simulink model "XY_Control"  (R2025b)
settings: Solver=FixedStepAuto  StartTime=0.0  StopTime=20  FixedStep=0.002  RelTol=1e-3  EnableMultiTasking=on
libraries: slpidlib x6, matrix_library x4, uavutilslib x1
settings Model: ExtModeTrigDuration=10000  Creator=plad  LastModifiedBy=David
settings SolverCC: AlgebraicLoopSolver=TrustRegion  PositivePriorityOrder=on
settings DataIOCC: ReturnWorkspaceOutputs=off
settings OptimizationCC: DefaultParameterBehavior=Inlined  EnhancedBackFolding=on  PassReuseOutputArgsAs=Individual arguments  ZeroExternalMemoryAtStartup=off  ZeroInternalMemoryAtStartup=off  MaxStackSize=64  OptimizeBlockOrder=speed  DifferentSizesBufferReuse=on  OptimizationCustomize=off  EfficientTunableParamExpr=on
settings DebuggingCC: ParameterTunabilityLossMsg=error  UnconnectedInputMsg=warning  UnconnectedOutputMsg=warning  UnconnectedLineMsg=warning  ArithmeticOperatorsInVariantConditions=warning
settings HardwareCC: ProdBitPerPointer=32.0  ProdBitPerSizeT=32.0  ProdBitPerPtrDiffT=32.0  ProdLargestAtomicFloat=None  ProdIntDivRoundTo=Undefined  ProdEndianess=Unspecified  ProdWordSize=32.0  ProdHWDeviceType=Generic->Unspecified (assume 32-bit Generic)
settings ModelReferenceCC: EnableRefExpFcnMdlSchedulingChecks=on
settings SFSimCC: SimUseLocalCustomCode=off  MATLABDynamicMemAlloc=off  CustomCodeUndefinedFunction=UseInterfaceOnly
settings RTWCC: SystemTargetFile=ert.tlc  TemplateMakefile=ert_default_tmf  RTWUseLocalCustomCode=off  TargetLang=C++  GPUComputeCapability=3.5  Description=Embedded Coder
settings CodeAppCC: ForceParamTrailComments=on  IgnoreCustomStorageClasses=off  OperatorAnnotations=on  SimulinkDataObjDesc=on  SFDataObjDesc=on  InsertBlockDesc=on
settings ERTTargetCC: ERTCustomFileTemplate=example_file_process.tlc
settings ConfigComp: CovMetricSettings=dswe

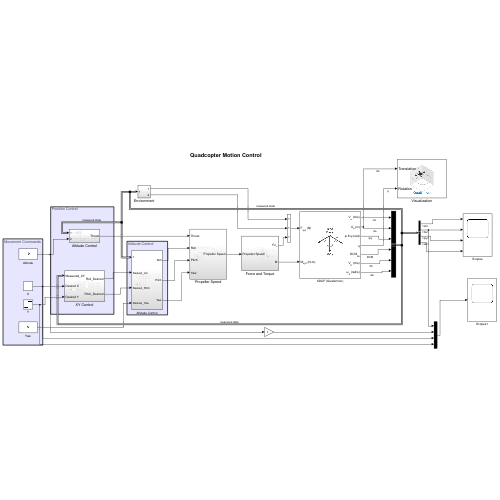
[thumbnail: Simulink's stored preview of the top-level diagram]
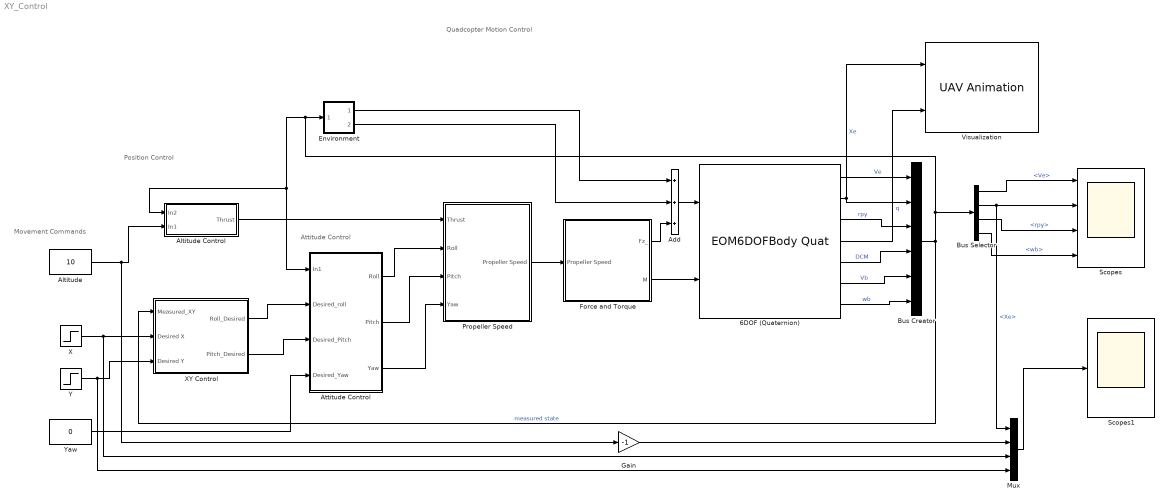
== system XY_Control ==
  note: Quadcopter Motion Control
  note: Attitude Control
  note: Position Control
  note: Movement Commands
  6DOF (Quaternion) : EOM6DOFBodyQuat
  Add : Sum  Inputs=+++
  Altitude : Constant  Value=10
  Altitude Control : Subsystem
  Attitude Control : Subsystem
  Bus Creator : BusCreator  Inputs=6
  Bus Selector : BusSelector  OutputSignals=Ve,Xe,rpy,wb
  Environment : Subsystem
  Force and Torque : Subsystem
  Gain : Gain  Gain=-1
  Mux : Mux
  Propeller Speed : Subsystem
  Scopes : Scope  NumInputPorts=4
      settings: ActiveDisplayYMinimum=-1  ActiveDisplayYMaximum=1
  Scopes1 : Scope
      settings: ActiveDisplayYMinimum=-65.352663287715231  ActiveDisplayYMaximum=14.57508700790809
  Visualization : uavutilslib/UAV Animation  NumUAV=1  DynamicUAVConfig=off  UAVType=Multirotor  UAVSize=1  UAVColor=[1 0 0]  UAVTrajectoryAlpha=1  InertialZDirection=Down  RotationFormat=Quaternion  DrawMarkers=off  SampleTime=-1
  X : Step  Time=3  After=4  SampleTime=0
  XY Control : Subsystem
  Y : Step  Time=3  After=8  SampleTime=0
  Yaw : Constant  Value=0
  wires:
  6DOF (Quaternion)/4 -> Visualization/2  "q"
  Altitude/1 -> Gain/1, Altitude Control/2(In1)
  X/1 -> Mux/3, XY Control/2(Desired X)
  Y/1 -> Mux/4, XY Control/3(Desired Y)
  XY Control/1(Roll_Desired) -> Attitude Control/2(Desired_roll)
  XY Control/2(Pitch_Desired) -> Attitude Control/3(Desired_Pitch)
  Yaw/1 -> Attitude Control/4(Desired_Yaw)
  Bus Creator/1 -> XY Control/1(Measured_XY), Attitude Control/1(In1), Altitude Control/1(In2), Environment/1(In1), Bus Selector/1  "measured state"
  Altitude Control/1(Thrust) -> Propeller Speed/1(Thrust)
  Attitude Control/1(Roll) -> Propeller Speed/2(Roll)
  Bus Selector/4 -> Scopes/4  "<wb>"
  Environment/1(Out1) -> Add/1
  Attitude Control/3(Yaw) -> Propeller Speed/4(Yaw)
  Attitude Control/2(Pitch) -> Propeller Speed/3(Pitch)
  Bus Selector/3 -> Scopes/3  "<rpy>"
  Bus Selector/1 -> Scopes/1  "<Ve>"
  Bus Selector/2 -> Scopes/2, Mux/1  "<Xe>"
  Environment/2(Out2) -> Add/2
  Propeller Speed/1(Propeller Speed) -> Force and Torque/1(Propeller Speed)
  Force and Torque/1(Fz_) -> Add/3
  6DOF (Quaternion)/2 -> Visualization/1, Bus Creator/2  "Xe"
  Add/1 -> 6DOF (Quaternion)/1
  Force and Torque/2(M) -> 6DOF (Quaternion)/2
  6DOF (Quaternion)/1 -> Bus Creator/1  "Ve"
  6DOF (Quaternion)/3 -> Bus Creator/3  "rpy"
  6DOF (Quaternion)/5 -> Bus Creator/4  "DCM"
  6DOF (Quaternion)/6 -> Bus Creator/5  "Vb"
  6DOF (Quaternion)/7 -> Bus Creator/6  "wb"
  Mux/1 -> Scopes1/1
  Gain/1 -> Mux/2

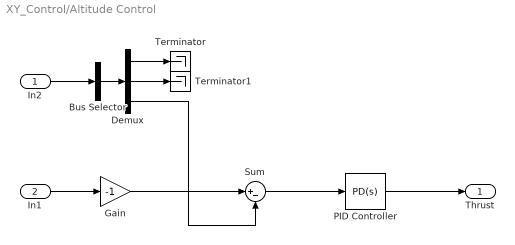
== system XY_Control/Altitude Control ==
  In2 : Inport
  In1 : Inport  Port=2
  Bus Selector : BusSelector  OutputSignals=Xe  OutputAsBus=on
  Demux : Demux  Outputs=3
  Gain : Gain  Gain=-1
  PID Controller : slpidlib/PID Controller  Controller=PD  Form=Parallel  TimeDomain=Continuous-time  UseExternalTs=off  SampleTime=-1  IntegratorMethod=Forward Euler  FilterMethod=Forward Euler  ControllerParametersSource=internal  P=1  I=1  UseKiTs=off  D=2  UseExternalDerivativeSource=off  N=100  UseFilter=on  TunerSelectOption=Transfer Function Based (PID Tuner App)  InitialConditionSource=internal  InitialConditionForIntegrator=0  InitialConditionForFilter=0  DifferentiatorICPrevScaledInput=0  ExternalReset=none  TrackingMode=off  Kt=1  LimitOutput=off  SatLimitsSource=internal  UpperSaturationLimit=inf  LowerSaturationLimit=-inf  LinearizeAsGain=on  AntiWindupMode=none  Kb=1  LimitIntegrator=off  UpperIntegratorSaturationLimit=inf  LowerIntegratorSaturationLimit=-inf  POutMin=[]  POutMax=[]  IOutMin=[]  IOutMax=[]  DOutMin=[]  DOutMax=[]  NOutMin=[]  NOutMax=[]  SumOutMin=[]  SumOutMax=[]  SaturationOutMin=[]  SaturationOutMax=[]  PParamMin=[]  PParamMax=[]  IParamMin=[]  IParamMax=[]  DParamMin=[]  DParamMax=[]  NParamMin=[]  NParamMax=[]  KbParamMin=[]  KbParamMax=[]  KtParamMin=[]  KtParamMax=[]  KbOutMin=[]  KbOutMax=[]  KtOutMin=[]  KtOutMax=[]  IntegratorOutMin=[]  IntegratorOutMax=[]  FilterOutMin=[]  FilterOutMax=[]  SumI1OutMin=[]  SumI1OutMax=[]  SumI2OutMin=[]  SumI2OutMax=[]  SumI3OutMin=[]  SumI3OutMax=[]  SumI4OutMin=[]  SumI4OutMax=[]  SumDOutMin=[]  SumDOutMax=[]  DifferentiatorOutMin=[]  DifferentiatorOutMax=[]  FilterDiffOutCoefMin=[]  FilterDiffOutCoefMax=[]  ReciprocalOutMin=[]  ReciprocalOutMax=[]  SumDenOutMin=[]  SumDenOutMax=[]  SumNumOutMin=[]  SumNumOutMax=[]  DivideOutMin=[]  DivideOutMax=[]  UdiffTsProdOutMin=[]  UdiffTsProdOutMax=[]  NTsProdOutMin=[]  NTsProdOutMax=[]  UintegralTsProdOutMin=[]  UintegralTsProdOutMax=[]  UngainTsProdOutMin=[]  UngainTsProdOutMax=[]  ClampingZeroOutDataTypeStr=Inherit: Inherit via back propagation  ClampingZeroOutMin=[]  ClampingZeroOutMax=[]  FilterDenConstantOutDataTypeStr=Inherit: Inherit via back propagation  FilterDenConstantOutMin=[]  FilterDenConstantOutMax=[]  PCopyOutDataTypeStr=Inherit: Inherit via back propagation  PCopyOutMin=[]  PCopyOutMax=[]  NCopyOutDataTypeStr=Inherit: Inherit via back propagation  NCopyOutMin=[]  NCopyOutMax=[]  IntegratorContinuousStateAttributes=''  IntegratorStateMustResolveToSignalObject=off  IntegratorRTWStateStorageClass=Auto  FilterContinuousStateAttributes=''  FilterStateMustResolveToSignalObject=off  FilterRTWStateStorageClass=Auto  ParallelPVariant=InternalParameters  IdealPVariant=Disabled  IVariant=Disabled  DVariant=InternalParameters  IntegratorVariant=Disabled  SatVariant=Disabled  AWVariant=Disabled  PCopyVariant=Disabled  TRVariant=Disabled  FdbkBlocksVariant=Forward  IdealPFdbkVariant=Disabled  SatFdbkVariant=Disabled  DerivativeFilterVariant=ContFilter  NVariant=InternalParameters  NCopyVariant=Disabled  FilterICVariant=InternalICsFilter  IntegratorICVariant=Disabled  ExternalResetVariant=Disabled  TRSumVariant=Passthrough  SumFdbkVariant=Disabled  SumVariant=Sum_PD  TsampFilterVariant=InternalTs  TsampNgainVariant=Passthrough  TsampIntegralVariant=Disabled_SignalSpec  ExternalSaturationOutDataTypeStr=Inherit: Same as second input  DerivativeSourceVariant=ErrorSignal  PreIntVariant=InternalPreInt
  Sum : Sum  Inputs=|+-
  Terminator : Terminator
  Terminator1 : Terminator
  Thrust : Outport
  wires:
  In2/1 -> Bus Selector/1
  Bus Selector/1 -> Demux/1
  Demux/2 -> Terminator1/1
  Demux/1 -> Terminator/1
  In1/1 -> Gain/1
  Demux/3 -> Sum/2
  Sum/1 -> PID Controller/1
  PID Controller/1 -> Thrust/1
  Gain/1 -> Sum/1

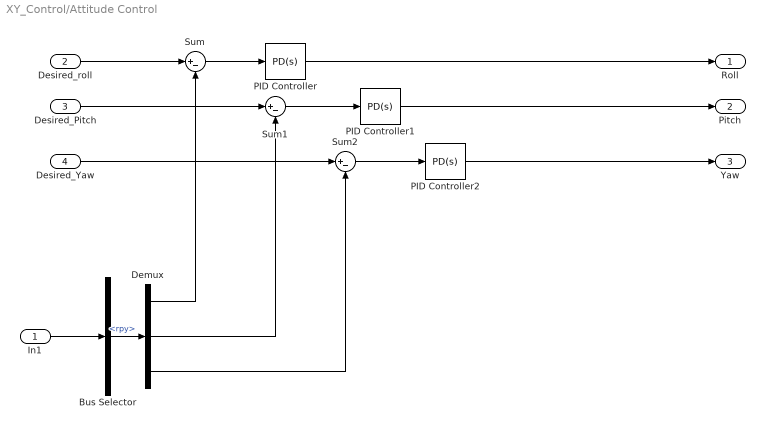
== system XY_Control/Attitude Control ==
  In1 : Inport
  Desired_roll : Inport  Port=2
  Desired_Pitch : Inport  Port=3
  Desired_Yaw : Inport  Port=4
  Bus Selector : BusSelector  OutputSignals=rpy
  Demux : Demux  Outputs=3
  PID Controller : slpidlib/PID Controller  Controller=PD  Form=Parallel  TimeDomain=Continuous-time  UseExternalTs=off  SampleTime=-1  IntegratorMethod=Forward Euler  FilterMethod=Forward Euler  ControllerParametersSource=internal  P=1  I=1  UseKiTs=off  D=2  UseExternalDerivativeSource=off  N=100  UseFilter=on  TunerSelectOption=Transfer Function Based (PID Tuner App)  InitialConditionSource=internal  InitialConditionForIntegrator=0  InitialConditionForFilter=0  DifferentiatorICPrevScaledInput=0  ExternalReset=none  TrackingMode=off  Kt=1  LimitOutput=off  SatLimitsSource=internal  UpperSaturationLimit=inf  LowerSaturationLimit=-inf  LinearizeAsGain=on  AntiWindupMode=none  Kb=1  LimitIntegrator=off  UpperIntegratorSaturationLimit=inf  LowerIntegratorSaturationLimit=-inf  POutMin=[]  POutMax=[]  IOutMin=[]  IOutMax=[]  DOutMin=[]  DOutMax=[]  NOutMin=[]  NOutMax=[]  SumOutMin=[]  SumOutMax=[]  SaturationOutMin=[]  SaturationOutMax=[]  PParamMin=[]  PParamMax=[]  IParamMin=[]  IParamMax=[]  DParamMin=[]  DParamMax=[]  NParamMin=[]  NParamMax=[]  KbParamMin=[]  KbParamMax=[]  KtParamMin=[]  KtParamMax=[]  KbOutMin=[]  KbOutMax=[]  KtOutMin=[]  KtOutMax=[]  IntegratorOutMin=[]  IntegratorOutMax=[]  FilterOutMin=[]  FilterOutMax=[]  SumI1OutMin=[]  SumI1OutMax=[]  SumI2OutMin=[]  SumI2OutMax=[]  SumI3OutMin=[]  SumI3OutMax=[]  SumI4OutMin=[]  SumI4OutMax=[]  SumDOutMin=[]  SumDOutMax=[]  DifferentiatorOutMin=[]  DifferentiatorOutMax=[]  FilterDiffOutCoefMin=[]  FilterDiffOutCoefMax=[]  ReciprocalOutMin=[]  ReciprocalOutMax=[]  SumDenOutMin=[]  SumDenOutMax=[]  SumNumOutMin=[]  SumNumOutMax=[]  DivideOutMin=[]  DivideOutMax=[]  UdiffTsProdOutMin=[]  UdiffTsProdOutMax=[]  NTsProdOutMin=[]  NTsProdOutMax=[]  UintegralTsProdOutMin=[]  UintegralTsProdOutMax=[]  UngainTsProdOutMin=[]  UngainTsProdOutMax=[]  ClampingZeroOutDataTypeStr=Inherit: Inherit via back propagation  ClampingZeroOutMin=[]  ClampingZeroOutMax=[]  FilterDenConstantOutDataTypeStr=Inherit: Inherit via back propagation  FilterDenConstantOutMin=[]  FilterDenConstantOutMax=[]  PCopyOutDataTypeStr=Inherit: Inherit via back propagation  PCopyOutMin=[]  PCopyOutMax=[]  NCopyOutDataTypeStr=Inherit: Inherit via back propagation  NCopyOutMin=[]  NCopyOutMax=[]  IntegratorContinuousStateAttributes=''  IntegratorStateMustResolveToSignalObject=off  IntegratorRTWStateStorageClass=Auto  FilterContinuousStateAttributes=''  FilterStateMustResolveToSignalObject=off  FilterRTWStateStorageClass=Auto  ParallelPVariant=InternalParameters  IdealPVariant=Disabled  IVariant=Disabled  DVariant=InternalParameters  IntegratorVariant=Disabled  SatVariant=Disabled  AWVariant=Disabled  PCopyVariant=Disabled  TRVariant=Disabled  FdbkBlocksVariant=Forward  IdealPFdbkVariant=Disabled  SatFdbkVariant=Disabled  DerivativeFilterVariant=ContFilter  NVariant=InternalParameters  NCopyVariant=Disabled  FilterICVariant=InternalICsFilter  IntegratorICVariant=Disabled  ExternalResetVariant=Disabled  TRSumVariant=Passthrough  SumFdbkVariant=Disabled  SumVariant=Sum_PD  TsampFilterVariant=InternalTs  TsampNgainVariant=Passthrough  TsampIntegralVariant=Disabled_SignalSpec  ExternalSaturationOutDataTypeStr=Inherit: Same as second input  DerivativeSourceVariant=ErrorSignal  PreIntVariant=InternalPreInt
  PID Controller1 : slpidlib/PID Controller  Controller=PD  Form=Parallel  TimeDomain=Continuous-time  UseExternalTs=off  SampleTime=-1  IntegratorMethod=Forward Euler  FilterMethod=Forward Euler  ControllerParametersSource=internal  P=1  I=1  UseKiTs=off  D=2  UseExternalDerivativeSource=off  N=100  UseFilter=on  TunerSelectOption=Transfer Function Based (PID Tuner App)  InitialConditionSource=internal  InitialConditionForIntegrator=0  InitialConditionForFilter=0  DifferentiatorICPrevScaledInput=0  ExternalReset=none  TrackingMode=off  Kt=1  LimitOutput=off  SatLimitsSource=internal  UpperSaturationLimit=inf  LowerSaturationLimit=-inf  LinearizeAsGain=on  AntiWindupMode=none  Kb=1  LimitIntegrator=off  UpperIntegratorSaturationLimit=inf  LowerIntegratorSaturationLimit=-inf  POutMin=[]  POutMax=[]  IOutMin=[]  IOutMax=[]  DOutMin=[]  DOutMax=[]  NOutMin=[]  NOutMax=[]  SumOutMin=[]  SumOutMax=[]  SaturationOutMin=[]  SaturationOutMax=[]  PParamMin=[]  PParamMax=[]  IParamMin=[]  IParamMax=[]  DParamMin=[]  DParamMax=[]  NParamMin=[]  NParamMax=[]  KbParamMin=[]  KbParamMax=[]  KtParamMin=[]  KtParamMax=[]  KbOutMin=[]  KbOutMax=[]  KtOutMin=[]  KtOutMax=[]  IntegratorOutMin=[]  IntegratorOutMax=[]  FilterOutMin=[]  FilterOutMax=[]  SumI1OutMin=[]  SumI1OutMax=[]  SumI2OutMin=[]  SumI2OutMax=[]  SumI3OutMin=[]  SumI3OutMax=[]  SumI4OutMin=[]  SumI4OutMax=[]  SumDOutMin=[]  SumDOutMax=[]  DifferentiatorOutMin=[]  DifferentiatorOutMax=[]  FilterDiffOutCoefMin=[]  FilterDiffOutCoefMax=[]  ReciprocalOutMin=[]  ReciprocalOutMax=[]  SumDenOutMin=[]  SumDenOutMax=[]  SumNumOutMin=[]  SumNumOutMax=[]  DivideOutMin=[]  DivideOutMax=[]  UdiffTsProdOutMin=[]  UdiffTsProdOutMax=[]  NTsProdOutMin=[]  NTsProdOutMax=[]  UintegralTsProdOutMin=[]  UintegralTsProdOutMax=[]  UngainTsProdOutMin=[]  UngainTsProdOutMax=[]  ClampingZeroOutDataTypeStr=Inherit: Inherit via back propagation  ClampingZeroOutMin=[]  ClampingZeroOutMax=[]  FilterDenConstantOutDataTypeStr=Inherit: Inherit via back propagation  FilterDenConstantOutMin=[]  FilterDenConstantOutMax=[]  PCopyOutDataTypeStr=Inherit: Inherit via back propagation  PCopyOutMin=[]  PCopyOutMax=[]  NCopyOutDataTypeStr=Inherit: Inherit via back propagation  NCopyOutMin=[]  NCopyOutMax=[]  IntegratorContinuousStateAttributes=''  IntegratorStateMustResolveToSignalObject=off  IntegratorRTWStateStorageClass=Auto  FilterContinuousStateAttributes=''  FilterStateMustResolveToSignalObject=off  FilterRTWStateStorageClass=Auto  ParallelPVariant=InternalParameters  IdealPVariant=Disabled  IVariant=Disabled  DVariant=InternalParameters  IntegratorVariant=Disabled  SatVariant=Disabled  AWVariant=Disabled  PCopyVariant=Disabled  TRVariant=Disabled  FdbkBlocksVariant=Forward  IdealPFdbkVariant=Disabled  SatFdbkVariant=Disabled  DerivativeFilterVariant=ContFilter  NVariant=InternalParameters  NCopyVariant=Disabled  FilterICVariant=InternalICsFilter  IntegratorICVariant=Disabled  ExternalResetVariant=Disabled  TRSumVariant=Passthrough  SumFdbkVariant=Disabled  SumVariant=Sum_PD  TsampFilterVariant=InternalTs  TsampNgainVariant=Passthrough  TsampIntegralVariant=Disabled_SignalSpec  ExternalSaturationOutDataTypeStr=Inherit: Same as second input  DerivativeSourceVariant=ErrorSignal  PreIntVariant=InternalPreInt
  PID Controller2 : slpidlib/PID Controller  Controller=PD  Form=Parallel  TimeDomain=Continuous-time  UseExternalTs=off  SampleTime=-1  IntegratorMethod=Forward Euler  FilterMethod=Forward Euler  ControllerParametersSource=internal  P=1  I=1  UseKiTs=off  D=2  UseExternalDerivativeSource=off  N=100  UseFilter=on  TunerSelectOption=Transfer Function Based (PID Tuner App)  InitialConditionSource=internal  InitialConditionForIntegrator=0  InitialConditionForFilter=0  DifferentiatorICPrevScaledInput=0  ExternalReset=none  TrackingMode=off  Kt=1  LimitOutput=off  SatLimitsSource=internal  UpperSaturationLimit=inf  LowerSaturationLimit=-inf  LinearizeAsGain=on  AntiWindupMode=none  Kb=1  LimitIntegrator=off  UpperIntegratorSaturationLimit=inf  LowerIntegratorSaturationLimit=-inf  POutMin=[]  POutMax=[]  IOutMin=[]  IOutMax=[]  DOutMin=[]  DOutMax=[]  NOutMin=[]  NOutMax=[]  SumOutMin=[]  SumOutMax=[]  SaturationOutMin=[]  SaturationOutMax=[]  PParamMin=[]  PParamMax=[]  IParamMin=[]  IParamMax=[]  DParamMin=[]  DParamMax=[]  NParamMin=[]  NParamMax=[]  KbParamMin=[]  KbParamMax=[]  KtParamMin=[]  KtParamMax=[]  KbOutMin=[]  KbOutMax=[]  KtOutMin=[]  KtOutMax=[]  IntegratorOutMin=[]  IntegratorOutMax=[]  FilterOutMin=[]  FilterOutMax=[]  SumI1OutMin=[]  SumI1OutMax=[]  SumI2OutMin=[]  SumI2OutMax=[]  SumI3OutMin=[]  SumI3OutMax=[]  SumI4OutMin=[]  SumI4OutMax=[]  SumDOutMin=[]  SumDOutMax=[]  DifferentiatorOutMin=[]  DifferentiatorOutMax=[]  FilterDiffOutCoefMin=[]  FilterDiffOutCoefMax=[]  ReciprocalOutMin=[]  ReciprocalOutMax=[]  SumDenOutMin=[]  SumDenOutMax=[]  SumNumOutMin=[]  SumNumOutMax=[]  DivideOutMin=[]  DivideOutMax=[]  UdiffTsProdOutMin=[]  UdiffTsProdOutMax=[]  NTsProdOutMin=[]  NTsProdOutMax=[]  UintegralTsProdOutMin=[]  UintegralTsProdOutMax=[]  UngainTsProdOutMin=[]  UngainTsProdOutMax=[]  ClampingZeroOutDataTypeStr=Inherit: Inherit via back propagation  ClampingZeroOutMin=[]  ClampingZeroOutMax=[]  FilterDenConstantOutDataTypeStr=Inherit: Inherit via back propagation  FilterDenConstantOutMin=[]  FilterDenConstantOutMax=[]  PCopyOutDataTypeStr=Inherit: Inherit via back propagation  PCopyOutMin=[]  PCopyOutMax=[]  NCopyOutDataTypeStr=Inherit: Inherit via back propagation  NCopyOutMin=[]  NCopyOutMax=[]  IntegratorContinuousStateAttributes=''  IntegratorStateMustResolveToSignalObject=off  IntegratorRTWStateStorageClass=Auto  FilterContinuousStateAttributes=''  FilterStateMustResolveToSignalObject=off  FilterRTWStateStorageClass=Auto  ParallelPVariant=InternalParameters  IdealPVariant=Disabled  IVariant=Disabled  DVariant=InternalParameters  IntegratorVariant=Disabled  SatVariant=Disabled  AWVariant=Disabled  PCopyVariant=Disabled  TRVariant=Disabled  FdbkBlocksVariant=Forward  IdealPFdbkVariant=Disabled  SatFdbkVariant=Disabled  DerivativeFilterVariant=ContFilter  NVariant=InternalParameters  NCopyVariant=Disabled  FilterICVariant=InternalICsFilter  IntegratorICVariant=Disabled  ExternalResetVariant=Disabled  TRSumVariant=Passthrough  SumFdbkVariant=Disabled  SumVariant=Sum_PD  TsampFilterVariant=InternalTs  TsampNgainVariant=Passthrough  TsampIntegralVariant=Disabled_SignalSpec  ExternalSaturationOutDataTypeStr=Inherit: Same as second input  DerivativeSourceVariant=ErrorSignal  PreIntVariant=InternalPreInt
  Sum : Sum  Inputs=|+-
  Sum1 : Sum  Inputs=|+-
  Sum2 : Sum  Inputs=|+-
  Roll : Outport
  Pitch : Outport  Port=2
  Yaw : Outport  Port=3
  wires:
  In1/1 -> Bus Selector/1
  Demux/3 -> Sum2/2
  Bus Selector/1 -> Demux/1  "<rpy>"
  Desired_roll/1 -> Sum/1
  Desired_Pitch/1 -> Sum1/1
  Desired_Yaw/1 -> Sum2/1
  Demux/1 -> Sum/2
  Demux/2 -> Sum1/2
  Sum/1 -> PID Controller/1
  PID Controller/1 -> Roll/1
  PID Controller1/1 -> Pitch/1
  Sum1/1 -> PID Controller1/1
  Sum2/1 -> PID Controller2/1
  PID Controller2/1 -> Yaw/1

== system XY_Control/Environment ==
  In1 : Inport
  Aerodynamic Drag : Subsystem
  Gravitational Force : Subsystem
  Out1 : Outport
  Out2 : Outport  Port=2
  wires:
  In1/1 -> Gravitational Force/1(In1), Aerodynamic Drag/1(In1)
  Aerodynamic Drag/1(Out1) -> Out1/1
  Gravitational Force/1(Out1) -> Out2/1

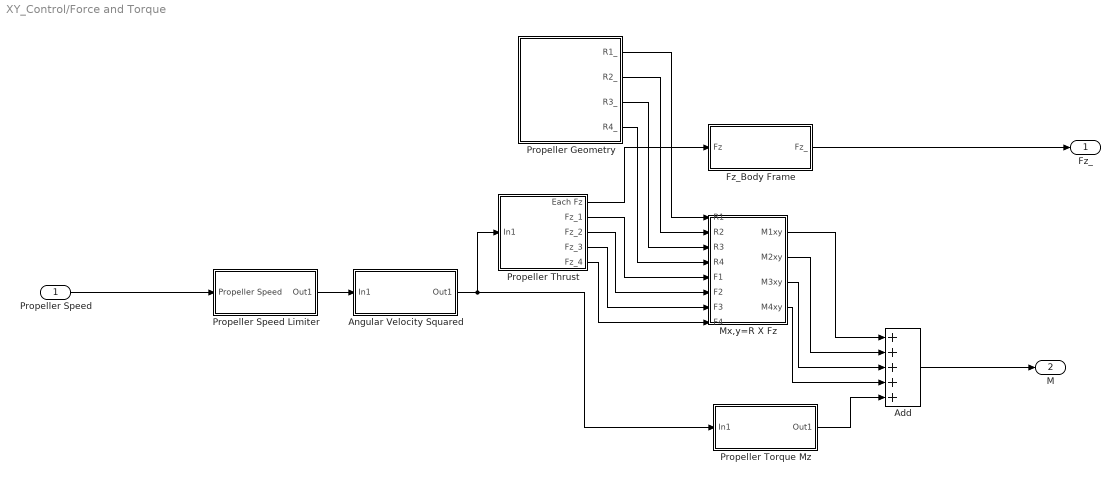
== system XY_Control/Force and Torque ==
  Propeller Speed : Inport
  Add : Sum  Inputs=+++++
  Angular Velocity Squared : Subsystem
  Fz_Body Frame : Subsystem
  Mx,y=R X Fz : Subsystem
  Propeller Geometry : Subsystem
  Propeller Speed Limiter : Subsystem
  Propeller Thrust : Subsystem
  Propeller Torque Mz : Subsystem
  Fz_ : Outport
  M : Outport  Port=2
  wires:
  Propeller Speed/1 -> Propeller Speed Limiter/1(Propeller Speed)
  Propeller Speed Limiter/1(Out1) -> Angular Velocity Squared/1(In1)
  Angular Velocity Squared/1(Out1) -> Propeller Torque Mz/1(In1), Propeller Thrust/1(In1)
  Add/1 -> M/1
  Propeller Torque Mz/1(Out1) -> Add/5
  Propeller Geometry/1(R1_) -> Mx,y=R X Fz/1(R1)
  Propeller Geometry/2(R2_) -> Mx,y=R X Fz/2(R2)
  Propeller Geometry/3(R3_) -> Mx,y=R X Fz/3(R3)
  Propeller Geometry/4(R4_) -> Mx,y=R X Fz/4(R4)
  Propeller Thrust/1(Each Fz) -> Fz_Body Frame/1(Fz)
  Propeller Thrust/2(Fz_1) -> Mx,y=R X Fz/5(F1)
  Propeller Thrust/3(Fz_2) -> Mx,y=R X Fz/6(F2)
  Propeller Thrust/4(Fz_3) -> Mx,y=R X Fz/7(F3)
  Propeller Thrust/5(Fz_4) -> Mx,y=R X Fz/8(F4)
  Fz_Body Frame/1(Fz_) -> Fz_/1
  Mx,y=R X Fz/1(M1xy) -> Add/1
  Mx,y=R X Fz/2(M2xy) -> Add/2
  Mx,y=R X Fz/3(M3xy) -> Add/3
  Mx,y=R X Fz/4(M4xy) -> Add/4

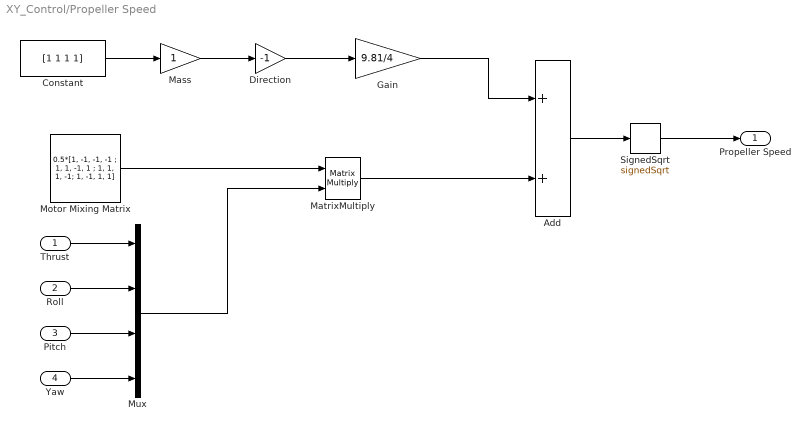
== system XY_Control/Propeller Speed ==
  Thrust : Inport
  Roll : Inport  Port=2
  Pitch : Inport  Port=3
  Yaw : Inport  Port=4
  Add : Sum
  Constant : Constant  Value=[1 1 1 1]
  Direction : Gain  Gain=-1
  Gain : Gain  Gain=9.81/4
  Mass : Gain
  MatrixMultiply : Product  Multiplication=Matrix(*)
  Motor Mixing Matrix : Constant  Value="0.5*[1, -1, -1, -1 ; 1, 1, -1, 1 ;   1, 1, 1, -1;  1, -1, 1, 1]"
  Mux : Mux
  SignedSqrt : Sqrt  Operator=signedSqrt  IntermediateResultsDataTypeStr=single
  Propeller Speed : Outport
  wires:
  Constant/1 -> Mass/1
  Mass/1 -> Direction/1
  Direction/1 -> Gain/1
  Gain/1 -> Add/1
  Thrust/1 -> Mux/1
  Roll/1 -> Mux/2
  Pitch/1 -> Mux/3
  Yaw/1 -> Mux/4
  Motor Mixing Matrix/1 -> MatrixMultiply/1
  Mux/1 -> MatrixMultiply/2
  MatrixMultiply/1 -> Add/2
  Add/1 -> SignedSqrt/1
  SignedSqrt/1 -> Propeller Speed/1

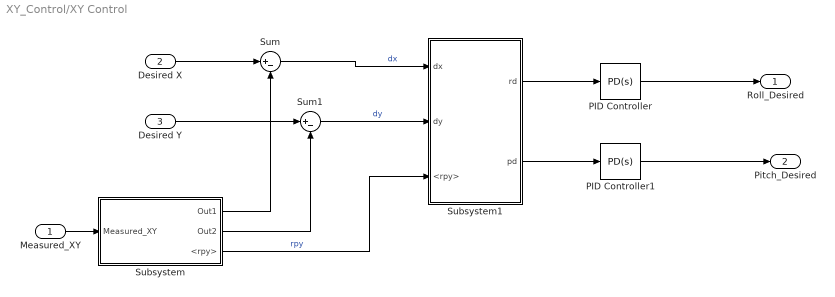
== system XY_Control/XY Control ==
  Measured_XY : Inport
  Desired X : Inport  Port=2
  Desired Y : Inport  Port=3
  PID Controller : slpidlib/PID Controller  Controller=PD  Form=Parallel  TimeDomain=Continuous-time  UseExternalTs=off  SampleTime=-1  IntegratorMethod=Forward Euler  FilterMethod=Forward Euler  ControllerParametersSource=internal  P=1  I=1  UseKiTs=off  D=2  UseExternalDerivativeSource=off  N=100  UseFilter=on  TunerSelectOption=Transfer Function Based (PID Tuner App)  InitialConditionSource=internal  InitialConditionForIntegrator=0  InitialConditionForFilter=0  DifferentiatorICPrevScaledInput=0  ExternalReset=none  TrackingMode=off  Kt=1  LimitOutput=on  SatLimitsSource=internal  UpperSaturationLimit=0.1  LowerSaturationLimit=-0.1  LinearizeAsGain=on  AntiWindupMode=none  Kb=1  LimitIntegrator=off  UpperIntegratorSaturationLimit=inf  LowerIntegratorSaturationLimit=-inf  POutMin=[]  POutMax=[]  IOutMin=[]  IOutMax=[]  DOutMin=[]  DOutMax=[]  NOutMin=[]  NOutMax=[]  SumOutMin=[]  SumOutMax=[]  SaturationOutMin=[]  SaturationOutMax=[]  PParamMin=[]  PParamMax=[]  IParamMin=[]  IParamMax=[]  DParamMin=[]  DParamMax=[]  NParamMin=[]  NParamMax=[]  KbParamMin=[]  KbParamMax=[]  KtParamMin=[]  KtParamMax=[]  KbOutMin=[]  KbOutMax=[]  KtOutMin=[]  KtOutMax=[]  IntegratorOutMin=[]  IntegratorOutMax=[]  FilterOutMin=[]  FilterOutMax=[]  SumI1OutMin=[]  SumI1OutMax=[]  SumI2OutMin=[]  SumI2OutMax=[]  SumI3OutMin=[]  SumI3OutMax=[]  SumI4OutMin=[]  SumI4OutMax=[]  SumDOutMin=[]  SumDOutMax=[]  DifferentiatorOutMin=[]  DifferentiatorOutMax=[]  FilterDiffOutCoefMin=[]  FilterDiffOutCoefMax=[]  ReciprocalOutMin=[]  ReciprocalOutMax=[]  SumDenOutMin=[]  SumDenOutMax=[]  SumNumOutMin=[]  SumNumOutMax=[]  DivideOutMin=[]  DivideOutMax=[]  UdiffTsProdOutMin=[]  UdiffTsProdOutMax=[]  NTsProdOutMin=[]  NTsProdOutMax=[]  UintegralTsProdOutMin=[]  UintegralTsProdOutMax=[]  UngainTsProdOutMin=[]  UngainTsProdOutMax=[]  ClampingZeroOutDataTypeStr=Inherit: Inherit via back propagation  ClampingZeroOutMin=[]  ClampingZeroOutMax=[]  FilterDenConstantOutDataTypeStr=Inherit: Inherit via back propagation  FilterDenConstantOutMin=[]  FilterDenConstantOutMax=[]  PCopyOutDataTypeStr=Inherit: Inherit via back propagation  PCopyOutMin=[]  PCopyOutMax=[]  NCopyOutDataTypeStr=Inherit: Inherit via back propagation  NCopyOutMin=[]  NCopyOutMax=[]  IntegratorContinuousStateAttributes=''  IntegratorStateMustResolveToSignalObject=off  IntegratorRTWStateStorageClass=Auto  FilterContinuousStateAttributes=''  FilterStateMustResolveToSignalObject=off  FilterRTWStateStorageClass=Auto  ParallelPVariant=InternalParameters  IdealPVariant=Disabled  IVariant=Disabled  DVariant=InternalParameters  IntegratorVariant=Disabled  SatVariant=Enabled  AWVariant=Disabled  PCopyVariant=Disabled  TRVariant=Disabled  FdbkBlocksVariant=Forward  IdealPFdbkVariant=Disabled  SatFdbkVariant=Disabled  DerivativeFilterVariant=ContFilter  NVariant=InternalParameters  NCopyVariant=Disabled  FilterICVariant=InternalICsFilter  IntegratorICVariant=Disabled  ExternalResetVariant=Disabled  TRSumVariant=Passthrough  SumFdbkVariant=Disabled  SumVariant=Sum_PD  TsampFilterVariant=InternalTs  TsampNgainVariant=Passthrough  TsampIntegralVariant=Disabled_SignalSpec  ExternalSaturationOutDataTypeStr=Inherit: Same as second input  DerivativeSourceVariant=ErrorSignal  PreIntVariant=InternalPreInt
  PID Controller1 : slpidlib/PID Controller  Controller=PD  Form=Parallel  TimeDomain=Continuous-time  UseExternalTs=off  SampleTime=-1  IntegratorMethod=Forward Euler  FilterMethod=Forward Euler  ControllerParametersSource=internal  P=1  I=1  UseKiTs=off  D=2  UseExternalDerivativeSource=off  N=100  UseFilter=on  TunerSelectOption=Frequency Response Based  InitialConditionSource=internal  InitialConditionForIntegrator=0  InitialConditionForFilter=0  DifferentiatorICPrevScaledInput=0  ExternalReset=none  TrackingMode=off  Kt=1  LimitOutput=on  SatLimitsSource=internal  UpperSaturationLimit=0.1  LowerSaturationLimit=-0.1  LinearizeAsGain=on  AntiWindupMode=none  Kb=1  LimitIntegrator=off  UpperIntegratorSaturationLimit=inf  LowerIntegratorSaturationLimit=-inf  POutMin=[]  POutMax=[]  IOutMin=[]  IOutMax=[]  DOutMin=[]  DOutMax=[]  NOutMin=[]  NOutMax=[]  SumOutMin=[]  SumOutMax=[]  SaturationOutMin=[]  SaturationOutMax=[]  PParamMin=[]  PParamMax=[]  IParamMin=[]  IParamMax=[]  DParamMin=[]  DParamMax=[]  NParamMin=[]  NParamMax=[]  KbParamMin=[]  KbParamMax=[]  KtParamMin=[]  KtParamMax=[]  KbOutMin=[]  KbOutMax=[]  KtOutMin=[]  KtOutMax=[]  IntegratorOutMin=[]  IntegratorOutMax=[]  FilterOutMin=[]  FilterOutMax=[]  SumI1OutMin=[]  SumI1OutMax=[]  SumI2OutMin=[]  SumI2OutMax=[]  SumI3OutMin=[]  SumI3OutMax=[]  SumI4OutMin=[]  SumI4OutMax=[]  SumDOutMin=[]  SumDOutMax=[]  DifferentiatorOutMin=[]  DifferentiatorOutMax=[]  FilterDiffOutCoefMin=[]  FilterDiffOutCoefMax=[]  ReciprocalOutMin=[]  ReciprocalOutMax=[]  SumDenOutMin=[]  SumDenOutMax=[]  SumNumOutMin=[]  SumNumOutMax=[]  DivideOutMin=[]  DivideOutMax=[]  UdiffTsProdOutMin=[]  UdiffTsProdOutMax=[]  NTsProdOutMin=[]  NTsProdOutMax=[]  UintegralTsProdOutMin=[]  UintegralTsProdOutMax=[]  UngainTsProdOutMin=[]  UngainTsProdOutMax=[]  ClampingZeroOutDataTypeStr=Inherit: Inherit via back propagation  ClampingZeroOutMin=[]  ClampingZeroOutMax=[]  FilterDenConstantOutDataTypeStr=Inherit: Inherit via back propagation  FilterDenConstantOutMin=[]  FilterDenConstantOutMax=[]  PCopyOutDataTypeStr=Inherit: Inherit via back propagation  PCopyOutMin=[]  PCopyOutMax=[]  NCopyOutDataTypeStr=Inherit: Inherit via back propagation  NCopyOutMin=[]  NCopyOutMax=[]  IntegratorContinuousStateAttributes=''  IntegratorStateMustResolveToSignalObject=off  IntegratorRTWStateStorageClass=Auto  FilterContinuousStateAttributes=''  FilterStateMustResolveToSignalObject=off  FilterRTWStateStorageClass=Auto  ParallelPVariant=InternalParameters  IdealPVariant=Disabled  IVariant=Disabled  DVariant=InternalParameters  IntegratorVariant=Disabled  SatVariant=Enabled  AWVariant=Disabled  PCopyVariant=Disabled  TRVariant=Disabled  FdbkBlocksVariant=Forward  IdealPFdbkVariant=Disabled  SatFdbkVariant=Disabled  DerivativeFilterVariant=ContFilter  NVariant=InternalParameters  NCopyVariant=Disabled  FilterICVariant=InternalICsFilter  IntegratorICVariant=Disabled  ExternalResetVariant=Disabled  TRSumVariant=Passthrough  SumFdbkVariant=Disabled  SumVariant=Sum_PD  TsampFilterVariant=InternalTs  TsampNgainVariant=Passthrough  TsampIntegralVariant=Disabled_SignalSpec  ExternalSaturationOutDataTypeStr=Inherit: Same as second input  DerivativeSourceVariant=ErrorSignal  PreIntVariant=InternalPreInt
  Subsystem : Subsystem
  Subsystem1 : Subsystem
  Sum : Sum  Inputs=|+-
  Sum1 : Sum  Inputs=|+-
  Roll_Desired : Outport
  Pitch_Desired : Outport  Port=2
  wires:
  Measured_XY/1 -> Subsystem/1(Measured_XY)
  Subsystem/1(Out1) -> Sum/2
  Subsystem/2(Out2) -> Sum1/2
  Desired X/1 -> Sum/1
  Desired Y/1 -> Sum1/1
  Sum/1 -> Subsystem1/1(dx)  "dx"
  Sum1/1 -> Subsystem1/2(dy)  "dy"
  Subsystem/3(<rpy>) -> Subsystem1/3(<rpy>)  "rpy"
  Subsystem1/2(pd) -> PID Controller1/1
  Subsystem1/1(rd) -> PID Controller/1
  PID Controller/1 -> Roll_Desired/1
  PID Controller1/1 -> Pitch_Desired/1

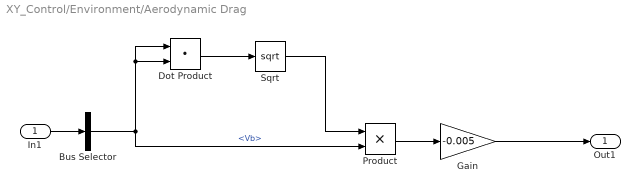
== system XY_Control/Environment/Aerodynamic Drag ==
  In1 : Inport
  Bus Selector : BusSelector  OutputSignals=Vb
  Dot Product : DotProduct  OutDataTypeStr=Inherit: Inherit via internal rule
  Gain : Gain  Gain=-0.005
  Product : Product
  Sqrt : Sqrt
  Out1 : Outport
  wires:
  In1/1 -> Bus Selector/1
  Bus Selector/1 -> Dot Product/1, Dot Product/2, Product/2  "<Vb>"
  Dot Product/1 -> Sqrt/1
  Sqrt/1 -> Product/1
  Product/1 -> Gain/1
  Gain/1 -> Out1/1

== system XY_Control/Environment/Gravitational Force ==
  In1 : Inport
  Gravitational Acceleration : Subsystem
  Mass : Gain
  Out1 : Outport
  wires:
  In1/1 -> Gravitational Acceleration/1(In1)
  Gravitational Acceleration/1(Out2) -> Mass/1
  Mass/1 -> Out1/1

== system XY_Control/Force and Torque/Angular Velocity Squared ==
  In1 : Inport
  Abs : Abs  SaturateOnIntegerOverflow=off
  Product : Product
  Out1 : Outport
  wires:
  Abs/1 -> Product/1
  Product/1 -> Out1/1
  In1/1 -> Product/2, Abs/1

== system XY_Control/Force and Torque/Fz_Body Frame ==
  Fz : Inport
  Sum of Elements : Sum  Inputs=+
  z-vector : Subsystem
  Fz_ : Outport
  wires:
  Fz/1 -> Sum of Elements/1
  z-vector/1(Fz_out) -> Fz_/1
  Sum of Elements/1 -> z-vector/1(Fz_in)

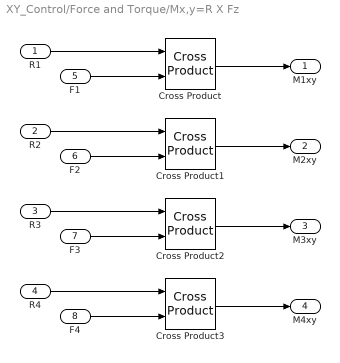
== system XY_Control/Force and Torque/Mx,y=R X Fz ==
  R1 : Inport
  R2 : Inport  Port=2
  R3 : Inport  Port=3
  R4 : Inport  Port=4
  F1 : Inport  Port=5
  F2 : Inport  Port=6
  F3 : Inport  Port=7
  F4 : Inport  Port=8
  Cross Product{,1..3} (4 alike) : matrix_library/Cross Product
  M1xy : Outport
  M2xy : Outport  Port=2
  M3xy : Outport  Port=3
  M4xy : Outport  Port=4
  wires:
  R1/1 -> Cross Product/1
  F1/1 -> Cross Product/2
  R2/1 -> Cross Product1/1
  F2/1 -> Cross Product1/2
  R3/1 -> Cross Product2/1
  F3/1 -> Cross Product2/2
  R4/1 -> Cross Product3/1
  F4/1 -> Cross Product3/2
  Cross Product/1 -> M1xy/1
  Cross Product1/1 -> M2xy/1
  Cross Product2/1 -> M3xy/1
  Cross Product3/1 -> M4xy/1

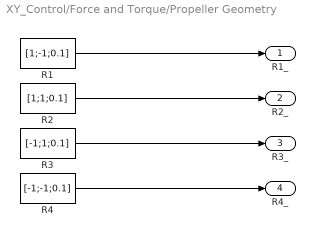
== system XY_Control/Force and Torque/Propeller Geometry ==
  R1 : Constant  Value=[1;-1;0.1]
  R2 : Constant  Value=[1;1;0.1]
  R3 : Constant  Value=[-1;1;0.1]
  R4 : Constant  Value=[-1;-1;0.1]
  R1_ : Outport
  R2_ : Outport  Port=2
  R3_ : Outport  Port=3
  R4_ : Outport  Port=4
  wires:
  R1/1 -> R1_/1
  R2/1 -> R2_/1
  R3/1 -> R3_/1
  R4/1 -> R4_/1

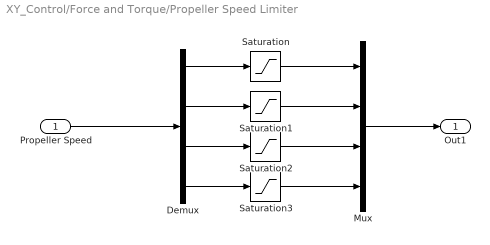
== system XY_Control/Force and Torque/Propeller Speed Limiter ==
  Propeller Speed : Inport
  Demux : Demux
  Mux : Mux
  Saturation{,1..3} (4 alike) : Saturate  UpperLimit=300  LowerLimit=-300
  Out1 : Outport
  wires:
  Propeller Speed/1 -> Demux/1
  Demux/1 -> Saturation/1
  Saturation/1 -> Mux/1
  Demux/2 -> Saturation1/1
  Demux/3 -> Saturation2/1
  Demux/4 -> Saturation3/1
  Saturation1/1 -> Mux/2
  Saturation2/1 -> Mux/3
  Saturation3/1 -> Mux/4
  Mux/1 -> Out1/1

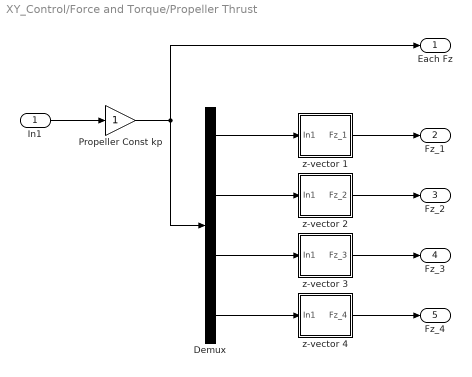
== system XY_Control/Force and Torque/Propeller Thrust ==
  In1 : Inport
  Demux : Demux
  Propeller Const kp : Gain
  z-vector 1 : Subsystem
  z-vector 2 : Subsystem
  z-vector 3 : Subsystem
  z-vector 4 : Subsystem
  Each Fz : Outport
  Fz_1 : Outport  Port=2
  Fz_2 : Outport  Port=3
  Fz_3 : Outport  Port=4
  Fz_4 : Outport  Port=5
  wires:
  In1/1 -> Propeller Const kp/1
  Propeller Const kp/1 -> Demux/1, Each Fz/1
  Demux/1 -> z-vector 1/1(In1)
  Demux/2 -> z-vector 2/1(In1)
  Demux/3 -> z-vector 3/1(In1)
  Demux/4 -> z-vector 4/1(In1)
  z-vector 1/1(Fz_1) -> Fz_1/1
  z-vector 2/1(Fz_2) -> Fz_2/1
  z-vector 3/1(Fz_3) -> Fz_3/1
  z-vector 4/1(Fz_4) -> Fz_4/1

== system XY_Control/Force and Torque/Propeller Torque Mz ==
  In1 : Inport
  Motor Torq Const km : Gain
  Subsystem : Subsystem
  Subsystem1 : Subsystem
  Out1 : Outport
  wires:
  In1/1 -> Motor Torq Const km/1
  Motor Torq Const km/1 -> Subsystem/1(In1)
  Subsystem/1(Out1) -> Subsystem1/1(In1)
  Subsystem1/1(Out1) -> Out1/1

== system XY_Control/XY Control/Subsystem ==
  Measured_XY : Inport
  Bus Selector : BusSelector  OutputSignals=Xe,rpy
  Demux : Demux  Outputs=3
  Terminator : Terminator
  Out1 : Outport
  Out2 : Outport  Port=2
  <rpy> : Outport  Port=3
  wires:
  Demux/3 -> Terminator/1
  Demux/2 -> Out2/1
  Measured_XY/1 -> Bus Selector/1
  Bus Selector/2 -> <rpy>/1  "<rpy>"
  Bus Selector/1 -> Demux/1  "<Xe>"
  Demux/1 -> Out1/1

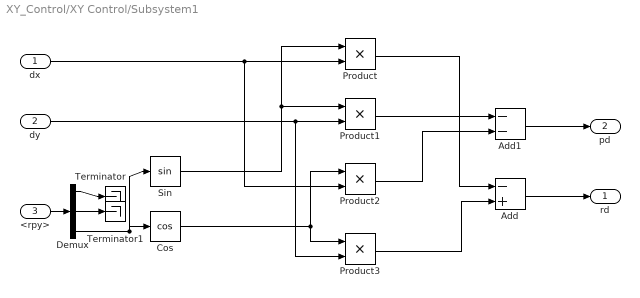
== system XY_Control/XY Control/Subsystem1 ==
  dx : Inport
  dy : Inport  Port=2
  <rpy> : Inport  Port=3
  Add : Sum  Inputs=-+
  Add1 : Sum  Inputs=--
  Cos : Trigonometry  Operator=cos
  Demux : Demux  Outputs=3
  Product{,1..3} (4 alike) : Product
  Sin : Trigonometry
  Terminator : Terminator
  Terminator1 : Terminator
  rd : Outport
  pd : Outport  Port=2
  wires:
  <rpy>/1 -> Demux/1
  Demux/1 -> Terminator/1
  Demux/2 -> Terminator1/1
  Demux/3 -> Cos/1, Sin/1
  Sin/1 -> Product/1, Product1/1
  dx/1 -> Product2/2, Product/2
  Product/1 -> Add/1
  Add/1 -> rd/1
  dy/1 -> Product3/2, Product1/2
  Product1/1 -> Add1/1
  Cos/1 -> Product3/1, Product2/1
  Product2/1 -> Add1/2
  Product3/1 -> Add/2
  Add1/1 -> pd/1

== system XY_Control/Environment/Gravitational Force/Gravitational Acceleration ==
  In1 : Inport
  Bus Selector1 : BusSelector  OutputSignals=DCM
  Constant2 : Constant  Value=[0;0;9.81]
  MatrixMultiply : Product  Multiplication=Matrix(*)
  Out2 : Outport
  wires:
  In1/1 -> Bus Selector1/1
  Bus Selector1/1 -> MatrixMultiply/1  "<DCM>"
  Constant2/1 -> MatrixMultiply/2
  MatrixMultiply/1 -> Out2/1

== system XY_Control/Force and Torque/Fz_Body Frame/z-vector ==
  Fz_in : Inport
  Constant : Constant  Value=[0;0;1]
  Product : Product
  Fz_out : Outport
  wires:
  Constant/1 -> Product/1
  Fz_in/1 -> Product/2
  Product/1 -> Fz_out/1

== system XY_Control/Force and Torque/Propeller Thrust/z-vector 1 ==
  In1 : Inport
  Product : Product
  az : Constant  Value=[0;0;1]
  Fz_1 : Outport
  wires:
  az/1 -> Product/1
  In1/1 -> Product/2
  Product/1 -> Fz_1/1

== system XY_Control/Force and Torque/Propeller Thrust/z-vector 2 ==
  In1 : Inport
  Product : Product
  az : Constant  Value=[0;0;1]
  Fz_2 : Outport
  wires:
  Product/1 -> Fz_2/1
  In1/1 -> Product/2
  az/1 -> Product/1

== system XY_Control/Force and Torque/Propeller Thrust/z-vector 3 ==
  In1 : Inport
  Product : Product
  az : Constant  Value=[0;0;1]
  Fz_3 : Outport
  wires:
  az/1 -> Product/1
  In1/1 -> Product/2
  Product/1 -> Fz_3/1

== system XY_Control/Force and Torque/Propeller Thrust/z-vector 4 ==
  In1 : Inport
  Product : Product
  az : Constant  Value=[0;0;1]
  Fz_4 : Outport
  wires:
  Product/1 -> Fz_4/1
  In1/1 -> Product/2
  az/1 -> Product/1

== system XY_Control/Force and Torque/Propeller Torque Mz/Subsystem ==
  In1 : Inport
  Constant : Constant  Value=[-1 1 -1 1]
  Product : Product
  Sum of Elements : Sum  Inputs=+
  Out1 : Outport
  wires:
  Constant/1 -> Product/1
  In1/1 -> Product/2
  Product/1 -> Sum of Elements/1
  Sum of Elements/1 -> Out1/1

== system XY_Control/Force and Torque/Propeller Torque Mz/Subsystem1 ==
  In1 : Inport
  Constant : Constant  Value=[0;0;1]
  Product : Product
  Out1 : Outport
  wires:
  Constant/1 -> Product/1
  In1/1 -> Product/2
  Product/1 -> Out1/1
